simulink model "SteeringCamera"  (R2025b)
settings: Solver=ode4  StartTime=0.0  StopTime=20  FixedStep=.001  RelTol=1e-3
undefined symbols (not defined in the file): cam_Ts, K_phi, K_rho, Kd_phi_out, Ki_phi_out, Kp_phi_in, Kp_phi_out, Kp_rho_in, m2ft, N_filt, phidot_max, sigma_phi, sigma_rho, V_bat, x0, y0
libraries: slpidlib x1
settings Model: Creator=jschw  LastModifiedBy=jschw

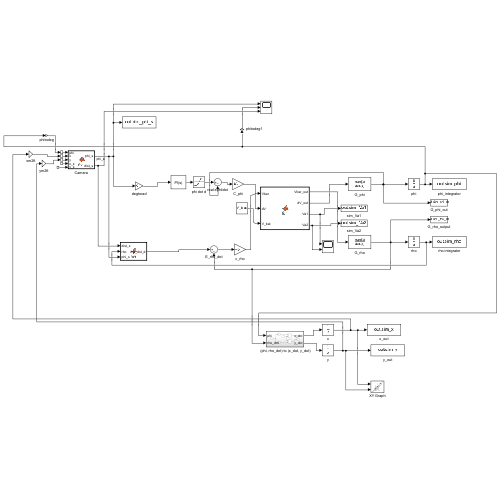
[thumbnail: Simulink's stored preview of the top-level diagram]
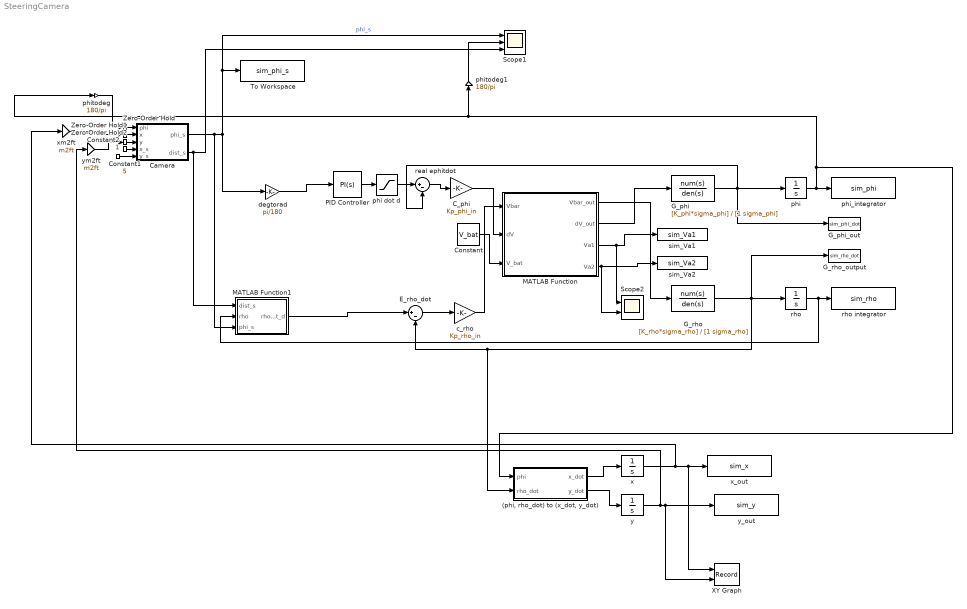
== system SteeringCamera ==
  " (phi, rho_dot) to (x_dot, y_dot)" : Subsystem
  C_phi : Gain  Gain=Kp_phi_in
  Camera : MATLAB Function  TreatAsAtomicUnit=on  SystemSampleTime=.2
  Constant : Constant  Value=V_bat
  Constant1 : Constant  Value=5
  Constant2 : Constant
  E_rho_dot : Sum  Inputs=|+-
  G_phi : TransferFcn  Numerator=[K_phi*sigma_phi]  Denominator=[1 sigma_phi]
  G_phi_out : ToWorkspace  VariableName=sim_phi_dot  SaveFormat=Timeseries  SampleTime=-1
  G_rho : TransferFcn  Numerator=[K_rho*sigma_rho]  Denominator=[1 sigma_rho]
  G_rho_output : ToWorkspace  VariableName=sim_rho_dot  SaveFormat=Timeseries  SampleTime=-1
  MATLAB Function : MATLAB Function  TreatAsAtomicUnit=on
  MATLAB Function1 : MATLAB Function  TreatAsAtomicUnit=on
  PID Controller : slpidlib/PID Controller  Controller=PI  Form=Parallel  TimeDomain=Continuous-time  UseExternalTs=off  SampleTime=-1  IntegratorMethod=Forward Euler  FilterMethod=Forward Euler  ControllerParametersSource=internal  P=Kp_phi_out  I=Ki_phi_out  UseKiTs=off  D=Kd_phi_out  UseExternalDerivativeSource=off  N=N_filt  UseFilter=on  TunerSelectOption=Transfer Function Based (PID Tuner App)  InitialConditionSource=internal  InitialConditionForIntegrator=0  InitialConditionForFilter=0  DifferentiatorICPrevScaledInput=0  ExternalReset=none  TrackingMode=off  Kt=1  LimitOutput=off  SatLimitsSource=internal  UpperSaturationLimit=inf  LowerSaturationLimit=-inf  LinearizeAsGain=on  AntiWindupMode=none  Kb=1  LimitIntegrator=off  UpperIntegratorSaturationLimit=inf  LowerIntegratorSaturationLimit=-inf  POutMin=[]  POutMax=[]  IOutMin=[]  IOutMax=[]  DOutMin=[]  DOutMax=[]  NOutMin=[]  NOutMax=[]  SumOutMin=[]  SumOutMax=[]  SaturationOutMin=[]  SaturationOutMax=[]  PParamMin=[]  PParamMax=[]  IParamMin=[]  IParamMax=[]  DParamMin=[]  DParamMax=[]  NParamMin=[]  NParamMax=[]  KbParamMin=[]  KbParamMax=[]  KtParamMin=[]  KtParamMax=[]  KbOutMin=[]  KbOutMax=[]  KtOutMin=[]  KtOutMax=[]  IntegratorOutMin=[]  IntegratorOutMax=[]  FilterOutMin=[]  FilterOutMax=[]  SumI1OutMin=[]  SumI1OutMax=[]  SumI2OutMin=[]  SumI2OutMax=[]  SumI3OutMin=[]  SumI3OutMax=[]  SumI4OutMin=[]  SumI4OutMax=[]  SumDOutMin=[]  SumDOutMax=[]  DifferentiatorOutMin=[]  DifferentiatorOutMax=[]  FilterDiffOutCoefMin=[]  FilterDiffOutCoefMax=[]  ReciprocalOutMin=[]  ReciprocalOutMax=[]  SumDenOutMin=[]  SumDenOutMax=[]  SumNumOutMin=[]  SumNumOutMax=[]  DivideOutMin=[]  DivideOutMax=[]  UdiffTsProdOutMin=[]  UdiffTsProdOutMax=[]  NTsProdOutMin=[]  NTsProdOutMax=[]  UintegralTsProdOutMin=[]  UintegralTsProdOutMax=[]  UngainTsProdOutMin=[]  UngainTsProdOutMax=[]  ClampingZeroOutDataTypeStr=Inherit: Inherit via back propagation  ClampingZeroOutMin=[]  ClampingZeroOutMax=[]  FilterDenConstantOutDataTypeStr=Inherit: Inherit via back propagation  FilterDenConstantOutMin=[]  FilterDenConstantOutMax=[]  PCopyOutDataTypeStr=Inherit: Inherit via back propagation  PCopyOutMin=[]  PCopyOutMax=[]  NCopyOutDataTypeStr=Inherit: Inherit via back propagation  NCopyOutMin=[]  NCopyOutMax=[]  IntegratorContinuousStateAttributes=''  IntegratorStateMustResolveToSignalObject=off  IntegratorRTWStateStorageClass=Auto  FilterContinuousStateAttributes=''  FilterStateMustResolveToSignalObject=off  FilterRTWStateStorageClass=Auto  ParallelPVariant=InternalParameters  IdealPVariant=Disabled  IVariant=InternalParameters  DVariant=Disabled  IntegratorVariant=Continuous  SatVariant=Disabled  AWVariant=Passthrough  PCopyVariant=Disabled  TRVariant=Disabled  FdbkBlocksVariant=Forward  IdealPFdbkVariant=Disabled  SatFdbkVariant=Disabled  DerivativeFilterVariant=Disabled  NVariant=Disabled  NCopyVariant=Disabled_SignalSpec  FilterICVariant=Disabled  IntegratorICVariant=InternalICs  ExternalResetVariant=Disabled  TRSumVariant=Passthrough  SumFdbkVariant=Disabled  SumVariant=Sum_PI  TsampFilterVariant=InternalTs  TsampNgainVariant=Passthrough  TsampIntegralVariant=Disabled_SignalSpec  ExternalSaturationOutDataTypeStr=Inherit: Same as second input  DerivativeSourceVariant=Disabled  PreIntVariant=InternalPreInt
  Scope1 : Scope  NumInputPorts=3
      settings: ActiveDisplayYMinimum=-195.1331606618167  ActiveDisplayYMaximum=120.43614199059992
  Scope2 : Scope  NumInputPorts=2
      settings: ActiveDisplayYMinimum=-7.3608867238318183  ActiveDisplayYMaximum=5.6267811820121061
  To Workspace : ToWorkspace  VariableName=sim_phi_s  SaveFormat=Timeseries  SampleTime=cam_Ts
  XY Graph : Record  NumPorts=2.0  FileSettingsInternal="{\"entries\":[{\"content\":{\"excelSettings\":{\"content\":{},\"type\":\"Streamout.ExcelSettings\"},\"parquetSettings\":{\"content\":{},\"type\":\"Streamout.ParquetSettings\"}},\"type\":\"Streamout.FileSettingStorage\",\"uuid\":\"\"}],\"packageUris\":[\"http:\\/\\/schema.mathworks.com\\/mf0\\/streamout_blocks\\/R2020a\"],\"version\":\"1.0\"}"  FrameSettings=[0, 0]  Layout=[1 1]  SignalsInternal="{\"entries\":[{\"content\":{\"signals\":[{\"content\":{\"blockPath\":[],\"dimensions\":[1],\"domain\":\"\",\"lineColor\":\"#fe330a\",\"lineWidth\":2,\"port\":1,\"sid\":[\"\"],\"signalID\":1,\"signalName\":\"x\"},\"type\":\"RecordBlkView.Signal\",\"uuid\":\"\"},{\"content\":{\"blockPath\":[],\"dimensions\":[1],\"domain\":\"\",\"lineColor\":\"#139fff\",\"plots\":[ 1 ],\"port\":2,\"sid\":[\"\"],\"signalID\":2,\"signalName\":\"y\"},\"type\":\"RecordBlkView.Signal\",\"uuid\":\"\"}]},\"type\":\"RecordBlkView.InputSignals\",\"uuid\":\"\"}],\"packageUris\":[\"http:\\/\\/schema.mathworks.com\\/mf0\\/streamout_blocks\\/R2020a\"],\"version\":\"1.0\"}"  VisualizationBindings="{\"xyplotplugin\":{\"info\":[{\"series\":[{\"bindingParametersList\":[{\"parameter\":\"Y-Axis\",\"signalID\":2,\"signalName\":\"y\"}],\"seriesID\":0}],\"subplotID\":1}]}}"  CompatibilityTag=XY
  Zero-Order Hold : ZeroOrderHold  SampleTime=cam_Ts
  Zero-Order Hold1 : ZeroOrderHold  SampleTime=cam_Ts
  Zero-Order Hold2 : ZeroOrderHold  SampleTime=cam_Ts
  c_rho : Gain  Gain=Kp_rho_in
  degtorad : Gain  Gain=pi/180
  phi : Integrator
  phi dot d : Saturate  UpperLimit=phidot_max  LowerLimit=-phidot_max
  phi_integrator : ToWorkspace  VariableName=sim_phi  SaveFormat=Timeseries  SampleTime=-1
  phitodeg : Gain  Gain=180/pi
  phitodeg1 : Gain  Gain=180/pi
  real ephitdot : Sum  Inputs=|+-
  rho : Integrator
  rho integrator : ToWorkspace  VariableName=sim_rho  SaveFormat=Timeseries  SampleTime=-1
  sim_Va1 : ToWorkspace  VariableName=sim_Va1  SaveFormat=Timeseries  SampleTime=-1
  sim_Va2 : ToWorkspace  VariableName=sim_Va2  SaveFormat=Timeseries  SampleTime=-1
  x : Integrator  InitialCondition=x0
  x_out : ToWorkspace  VariableName=sim_x  SaveFormat=Timeseries  SampleTime=-1
  xm2ft : Gain  Gain=m2ft
  y : Integrator  InitialCondition=y0
  y_out : ToWorkspace  VariableName=sim_y  SaveFormat=Timeseries  SampleTime=-1
  ym2ft : Gain  Gain=m2ft
  wires:
  E_rho_dot/1 -> c_rho/1
  c_rho/1 -> MATLAB Function/1(Vbar)
  Constant/1 -> MATLAB Function/3(V_bat)
  C_phi/1 -> MATLAB Function/2(dV)
  MATLAB Function/1(Vbar_out) -> G_rho/1
  MATLAB Function/2(dV_out) -> G_phi/1
  MATLAB Function/3(Va1) -> Scope2/1, sim_Va1/1
  MATLAB Function/4(Va2) -> Scope2/2, sim_Va2/1
  PID Controller/1 -> phi dot d/1
  phi dot d/1 -> real ephitdot/1
  real ephitdot/1 -> C_phi/1
  G_phi/1 -> real ephitdot/2, G_phi_out/1, phi/1
  rho/1 -> MATLAB Function1/2(rho), rho integrator/1
  G_rho/1 -> " (phi, rho_dot) to (x_dot, y_dot)"/2(rho_dot), E_rho_dot/2, G_rho_output/1, rho/1
  " (phi, rho_dot) to (x_dot, y_dot)"/2(y_dot) -> y/1
  " (phi, rho_dot) to (x_dot, y_dot)"/1(x_dot) -> x/1
  x/1 -> xm2ft/1, XY Graph/1, x_out/1
  y/1 -> ym2ft/1, XY Graph/2, y_out/1
  Zero-Order Hold/1 -> Camera/1(phi)
  Zero-Order Hold1/1 -> Camera/2(x)
  Zero-Order Hold2/1 -> Camera/3(y)
  Constant2/1 -> Camera/5(y_s)
  Constant1/1 -> Camera/4(x_s)
  xm2ft/1 -> Zero-Order Hold1/1
  ym2ft/1 -> Zero-Order Hold2/1
  phitodeg/1 -> Zero-Order Hold/1
  Camera/1(phi_s) -> MATLAB Function1/3(phi_s), degtorad/1, Scope1/1, To Workspace/1  "phi_s"
  degtorad/1 -> PID Controller/1
  MATLAB Function1/1(rho_dot_d) -> E_rho_dot/1
  phi/1 -> " (phi, rho_dot) to (x_dot, y_dot)"/1(phi), phitodeg1/1, phitodeg/1, phi_integrator/1
  Camera/2(dist_s) -> MATLAB Function1/1(dist_s), Scope1/3
  phitodeg1/1 -> Scope1/2

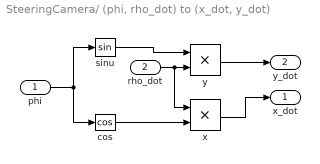
== system SteeringCamera/ (phi, rho_dot) to (x_dot, y_dot) ==
  phi : Inport
  rho_dot : Inport  Port=2
  cos : Trigonometry  Operator=cos
  sinu : Trigonometry
  x : Product
  y : Product
  x_dot : Outport
  y_dot : Outport  Port=2
  wires:
  rho_dot/1 -> x/1, y/2
  phi/1 -> cos/1, sinu/1
  sinu/1 -> y/1
  cos/1 -> x/2
  x/1 -> x_dot/1
  y/1 -> y_dot/1

== matlab function SteeringCamera/MATLAB Function ==
  data: Vbar input; Vbar_out output; dV input; V_bat input; dV_out output; Va1 output; Va2 output
function [Vbar_out, dV_out, Va1, Va2] = fcn(Vbar, dV, V_bat)
% Same saturation as SteeringInnerLoopTest.ino: scale both wheels
% together so the forward/turn ratio is kept
Va1 = (Vbar + dV)/2;
Va2 = (Vbar - dV)/2;
m = max(abs(Va1), abs(Va2));
if m > V_bat
    Va1 = Va1*V_bat/m;
    Va2 = Va2*V_bat/m;
end
Vbar_out = Va1 + Va2;
dV_out   = Va1 - Va2;

== matlab function SteeringCamera/Camera ==
  data: phi input; phi_s output; x input; y input; x_s input; y_s input; dist_s output
function [phi_s, dist_s] = fcn(phi,x,y,x_s,y_s)
%#codegen
% UPDATED camera block for Demo 2: simulates the Pi seeing ONE ArUco marker
% instead of a tape line. Same inputs as the original block, so no rewiring:
%   phi       robot heading, degrees (+ = left / CCW)
%   x, y      robot position, feet
%   x_s, y_s  MARKER position, feet. Set the two Constant blocks to single
%             numbers, e.g. x_s = 5, y_s = 0 (if they are still vectors, the
%             last point is used as the marker).
% Outputs:
%   phi_s     angle from the heading to the marker, degrees, + = left (0 if not seen)
%   dist_s    camera-to-marker distance, feet (0 if not seen). NEW output port:
%             wire it to a Scope / To Workspace, or leave it unconnected.
%
% Change these to simulate different situations:
angle_of_view = 53.5;   % deg, full field of view (same as the original block)
max_range     = 8;      % ft, farther than this the 2 in marker can't be decoded
cam_offset    = 0.33;   % ft (about 0.10 m) camera ahead of the wheel axle
noise_deg     = 0.0;    % deg, angle noise (std dev), 0 = perfect
noise_ft      = 0.0;    % ft, distance noise (std dev), 0 = perfect
% Frame rate = this block's sample time (0.2 s = 5 fps).
 
x_m = x_s(end);
y_m = y_s(end);
 
% Camera sits ahead of the center of rotation along the heading
ph = phi*pi/180;
xc = x + cam_offset*cos(ph);
yc = y + cam_offset*sin(ph);
 
% Marker in the robot's frame
dx = x_m - xc;
dy = y_m - yc;
fwd  =  cos(ph)*dx + sin(ph)*dy;   % ahead
left = -sin(ph)*dx + cos(ph)*dy;   % to the left
 
phi_s  = atan2(left, fwd)*180/pi;
dist_s = sqrt(dx^2 + dy^2);
 
% Seen only if in front, inside the field of view, and within range
if fwd > 0 && abs(phi_s) < angle_of_view/2 && dist_s < max_range
    phi_s  = phi_s  + noise_deg*randn;
    dist_s = dist_s + noise_ft*randn;
else
    phi_s  = 0;
    dist_s = 0;
end
end
 
% ======================================================================
% ORIGINAL tape-line camera code (commented out, kept for reference)
% ======================================================================
% function phi_s = fcn(phi,x,y,x_s,y_s)
% %#codegen
% %
% % Simulation of Camera with line detection
% % phi - angle of robot in degrees
% % x - x position of robot in feet
% % y - y position of robot in feet
% % x_s - vector of x coordinates for line to be detected (in feet)
% % y_s - vector of y coordinates for line to be detected (in feet)
% %
% %
% 
% % change show_image to 1 to see camera image during simulation
% show_image=0;
% %
% % number of horizontal and vertical pixels
% %
% h_pix = 740;
% v_pix = 480;
% %
% % pixel_check is the row of the image to check for the line (origin of
% % camera image is upper right
% % 
% pixel_check = v_pix*4/5;
% %
% % meters to feet conversion
% %
% mtof = 3.28;
% % f is focal length 
% %
% f = .0036; %m
% f = mtof*f; % convert to feet
% %
% % sensor image area
% %
% image_w = .00376; % m
% image_h = .00274; % m
% image_w = image_w*mtof; % convert to feet
% image_h = image_h*mtof; % convert to feet
% %
% % h is height of the camera 
% %
% h = 0.1; % m
% h = h*mtof; % convert to feet
% %
% % angle of view is from center to edge of camrea in radians
% %
% angle_of_view=53.5; % degrees
% 
% %
% % interpolate between line points
% %
% x_s = interp1q((1:length(x_s))',x_s,(1:.01:length(x_s))');
% y_s = interp1q((1:length(y_s))',y_s,(1:.01:length(y_s))');
% %
% % translate points to camera origin
% % 
% tape=[x_s,y_s]';
% % figure
% % plot(tape(1,:),tape(2,:),'*')
% % axis([-5 5 -5 5])
% 
% tape = tape - [x;y]*ones(1,size(tape,2));
% % figure
% % plot(tape(1,:),tape(2,:),'*')
% % axis([-5 5 -5 5])
% %
% % find points that are in the angle of view
% %
% angle = (180/pi)*acos(([cos(phi*pi/180) sin(phi*pi/180)]*tape)./sqrt(sum(tape.^2)));
% index=find(angle<angle_of_view/2 & angle>-angle_of_view/2);
% if isempty(index)
%     disp('Tape not visible to the robot')
%     phi_s = 0;
%     return
% end;
% tape=tape(:,index);
% % figure
% % plot(tape(1,:),tape(2,:),'*')
% % hold on
% % fill(v_c(1,:),v_c(2,:),'y')
% % title('visible points')
% % axis([-5 5 -5 5])
% %
% % rotate points so straight ahead is along x axis
% %
% tapenorm=[cos(phi*pi/180) sin(phi*pi/180);-sin(phi*pi/180) cos(phi*pi/180)]*tape;
% %
% % map onto film coordinates
% %
% image = [(f./tapenorm(1,:)).*(-tapenorm(2,:));
%     (f./tapenorm(1,:)).*(-h*ones(1,size(tapenorm,2)))];
% % figure
% % plot(image(1,:),image(2,:),'*')
% % axis([-image_w/2 image_w/2 -image_h/2 image_h/2])
% 
% %
% % map onto pixel coordinates
% %
% pixel = [0; v_pix]*ones(1,size(image,2)) + diag([h_pix/image_w -v_pix/image_h])*image+[h_pix/2; -v_pix/2]*ones(1,size(image,2));
% if (show_image)
%  figure(1)
%  plot(pixel(1,:),pixel(2,:),'*')
%  set(gca, 'YDir','reverse')
%  hold on
%  plot([0 h_pix],[pixel_check pixel_check],'r-')
%  axis([0 h_pix 0 v_pix])
%  hold off
%  title('Robot camera view set show_image=0 to turn off and speed up simulation','interpreter','none')
% end;
% 
% 
% %
% % find point on horizontal line at pixel number pixel_check
% %
% checkpoints= find(pixel(2,:)>=pixel_check);
% if ~isempty(checkpoints)
%     [m,index]=min(pixel(2,checkpoints));  
%     if abs(pixel(2,index)-pixel_check)>10,
%         disp(['no point visible near row ',int2str(pixel_check)])
%         phi_s = 0;
%         return
%     end;
% else
%     disp(['no point visible near row ',int2str(pixel_check)])
%     phi_s = 0;
%     return
% end;
% 
% 
% phi_s = -(pixel(1,index)-h_pix/2)*angle_of_view/h_pix;

== matlab function SteeringCamera/MATLAB Function1 ==
  settings: updateMethod=DISCRETE  sampleTime=.01
  data: dist_s input; rho_dot_d output; rho input; phi_s input
function rho_dot_d = fcn(dist_s, rho, phi_s)
% Turn in place until centered, take the distance once, then drive on encoders
persistent rho_goal
if isempty(rho_goal), rho_goal = NaN; end
stop_ft = 1.0; cam_ft = 0.33; Kp = 6; vmax = 0.5;
align_deg = 2;                       % same as AlignTol on the Arduino
if isnan(rho_goal) && dist_s > 0 && abs(phi_s) < align_deg
    rho_goal = rho + (dist_s + cam_ft - stop_ft)*0.3048;   % m
end
if isnan(rho_goal)
    rho_dot_d = 0;                   % still turning (or not seen): hold position
else
    rho_dot_d = min(max(Kp*(rho_goal - rho), -vmax), vmax);
end
